simulink model "system_model"  (R2025b)
settings: Solver=FixedStepAuto  StartTime=0.0  StopTime=10  FixedStep=t_s  RelTol=1e-3
values from neighbouring files (symbols this model uses):
  D = Cpid.Kd    [system_init.m]
  denom = [I*L I*R (L*c + k_f*k_e*r^2)  R*c]    [system_init.m]
  I_ = Cpid.Ki    [system_init.m]
  k_enc = 4096 / (2 * pi)    (= 651.898646904)    [system_init.m]
  N = 1/Cpid.Tf    [system_init.m]
  nom = r*k_f    (= 0.73794)    [system_init.m]
  P = Cpid.Kp    [system_init.m]
  r_2 = r    (= 0.1004)    [system_init.m]
  t_s = 0.0005    [system_init.m]
  V_max = 60    [system_init.m]
libraries: slpidlib x1
settings Model: Creator=KnaZ  LastModifiedBy=KnaZ

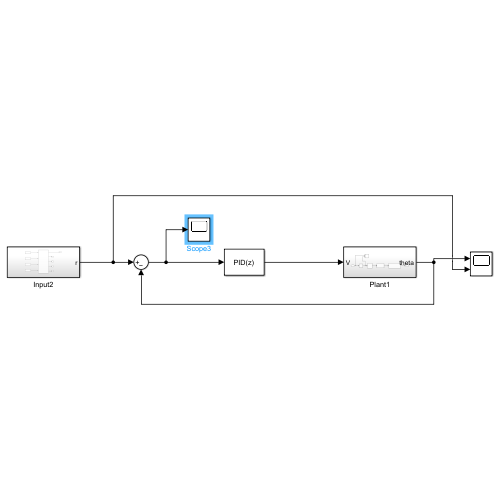
[thumbnail: Simulink's stored preview of the top-level diagram]
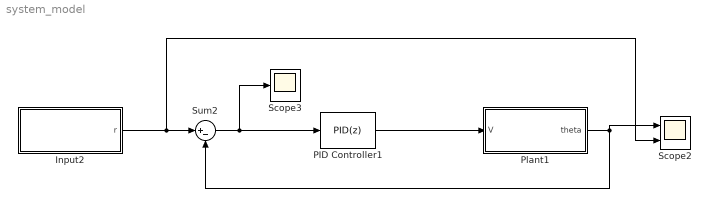
== system system_model ==
  Input2 : Subsystem
  PID Controller1 : slpidlib/PID Controller  Controller=PID  Form=Ideal  TimeDomain=Discrete-time  UseExternalTs=off  SampleTime=t_s  IntegratorMethod=Forward Euler  FilterMethod=Forward Euler  ControllerParametersSource=internal  P=P/10  I=I_  UseKiTs=off  D=D  UseExternalDerivativeSource=off  N=N  UseFilter=on  TunerSelectOption=Transfer Function Based (PID Tuner App)  InitialConditionSource=internal  InitialConditionForIntegrator=0  InitialConditionForFilter=0  DifferentiatorICPrevScaledInput=0  ExternalReset=none  TrackingMode=off  Kt=I_  LimitOutput=off  SatLimitsSource=internal  UpperSaturationLimit=60  LowerSaturationLimit=-60  LinearizeAsGain=off  AntiWindupMode=clamping  Kb=1  LimitIntegrator=off  UpperIntegratorSaturationLimit=inf  LowerIntegratorSaturationLimit=-inf  POutMin=[]  POutMax=[]  IOutMin=[]  IOutMax=[]  DOutMin=[]  DOutMax=[]  NOutMin=[]  NOutMax=[]  SumOutMin=[]  SumOutMax=[]  SaturationOutMin=[]  SaturationOutMax=[]  PParamMin=[]  PParamMax=[]  IParamMin=[]  IParamMax=[]  DParamMin=[]  DParamMax=[]  NParamMin=[]  NParamMax=[]  KbParamMin=[]  KbParamMax=[]  KtParamMin=[]  KtParamMax=[]  KbOutMin=[]  KbOutMax=[]  KtOutMin=[]  KtOutMax=[]  IntegratorOutMin=[]  IntegratorOutMax=[]  FilterOutMin=[]  FilterOutMax=[]  SumI1OutMin=[]  SumI1OutMax=[]  SumI2OutMin=[]  SumI2OutMax=[]  SumI3OutMin=[]  SumI3OutMax=[]  SumI4OutMin=[]  SumI4OutMax=[]  SumDOutMin=[]  SumDOutMax=[]  DifferentiatorOutMin=[]  DifferentiatorOutMax=[]  FilterDiffOutCoefMin=[]  FilterDiffOutCoefMax=[]  ReciprocalOutMin=[]  ReciprocalOutMax=[]  SumDenOutMin=[]  SumDenOutMax=[]  SumNumOutMin=[]  SumNumOutMax=[]  DivideOutMin=[]  DivideOutMax=[]  UdiffTsProdOutMin=[]  UdiffTsProdOutMax=[]  NTsProdOutMin=[]  NTsProdOutMax=[]  UintegralTsProdOutMin=[]  UintegralTsProdOutMax=[]  UngainTsProdOutMin=[]  UngainTsProdOutMax=[]  ClampingZeroOutDataTypeStr=Inherit: Inherit via back propagation  ClampingZeroOutMin=[]  ClampingZeroOutMax=[]  FilterDenConstantOutDataTypeStr=Inherit: Inherit via back propagation  FilterDenConstantOutMin=[]  FilterDenConstantOutMax=[]  PCopyOutDataTypeStr=Inherit: Inherit via back propagation  PCopyOutMin=[]  PCopyOutMax=[]  NCopyOutDataTypeStr=Inherit: Inherit via back propagation  NCopyOutMin=[]  NCopyOutMax=[]  IntegratorContinuousStateAttributes=''  IntegratorStateMustResolveToSignalObject=off  IntegratorRTWStateStorageClass=Auto  FilterContinuousStateAttributes=''  FilterStateMustResolveToSignalObject=off  FilterRTWStateStorageClass=Auto  ParallelPVariant=Passthrough  IdealPVariant=InternalParameters  IVariant=InternalParameters  DVariant=InternalParameters  IntegratorVariant=Discrete  SatVariant=Disabled  AWVariant=Passthrough  PCopyVariant=Disabled  TRVariant=Disabled  FdbkBlocksVariant=Forward  IdealPFdbkVariant=Disabled  SatFdbkVariant=Disabled  DerivativeFilterVariant=ForwardEulerFilter  NVariant=InternalParameters  NCopyVariant=Disabled  FilterICVariant=InternalICsFilter  IntegratorICVariant=InternalICs  ExternalResetVariant=Disabled  TRSumVariant=Passthrough  SumFdbkVariant=Disabled  SumVariant=Sum_PID  TsampFilterVariant=InternalTs  TsampNgainVariant=Passthrough  TsampIntegralVariant=Disabled_SignalSpec  ExternalSaturationOutDataTypeStr=Inherit: Same as second input  DerivativeSourceVariant=ErrorSignal  PreIntVariant=InternalPreInt
  Plant1 : Subsystem
  Scope2 : Scope  NumInputPorts=2
      settings: ActiveDisplayYMinimum=-0.020443518010116426  ActiveDisplayYMaximum=-0.0090093721690085588
  Scope3 : Scope
      settings: ActiveDisplayYMinimum=-0.0045939575455967042  ActiveDisplayYMaximum=0.0022798434903788887  DataLoggingVariableName=ScopeData2
  Sum2 : Sum  Inputs=|+-
  wires:
  Input2/1(r) -> Scope2/2, Sum2/1
  Plant1/1(theta) -> Scope2/1, Sum2/2
  PID Controller1/1 -> Plant1/1(V)
  Sum2/1 -> Scope3/1, PID Controller1/1

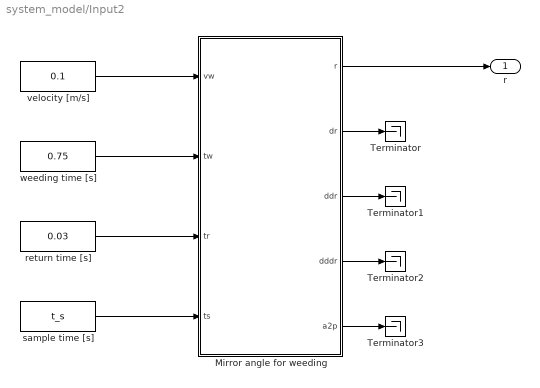
== system system_model/Input2 ==
  Mirror angle for weeding : MATLAB Function  TreatAsAtomicUnit=on
  Terminator{,1..3} (4 alike) : Terminator
  return time [s] : Constant  Value=0.03  SampleTime=t_s
  sample time [s] : Constant  Value=t_s  SampleTime=t_s
  velocity [m/s] : Constant  Value=0.1  SampleTime=t_s
  weeding time [s] : Constant  Value=0.75  SampleTime=t_s
  r : Outport
  wires:
  Mirror angle for weeding/3(ddr) -> Terminator1/1
  Mirror angle for weeding/4(dddr) -> Terminator2/1
  Mirror angle for weeding/1(r) -> r/1
  sample time [s]/1 -> Mirror angle for weeding/4(ts)
  Mirror angle for weeding/2(dr) -> Terminator/1
  return time [s]/1 -> Mirror angle for weeding/3(tr)
  weeding time [s]/1 -> Mirror angle for weeding/2(tw)
  velocity [m/s]/1 -> Mirror angle for weeding/1(vw)
  Mirror angle for weeding/5(a2p) -> Terminator3/1

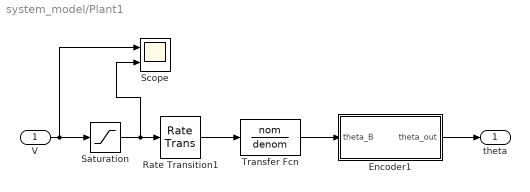
== system system_model/Plant1 ==
  V : Inport
  Encoder1 : Subsystem
  Rate Transition1 : RateTransition  OutPortSampleTime=0
  Saturation : Saturate  UpperLimit=V_max  LowerLimit=-V_max
  Scope : Scope  NumInputPorts=2
      settings: ActiveDisplayYMinimum=-94.384761555803735  ActiveDisplayYMaximum=107.07366746963213  DataLoggingVariableName=ScopeData3
  Transfer Fcn : TransferFcn  Numerator=nom  Denominator=denom
  theta : Outport
  wires:
  Encoder1/1(theta_out) -> theta/1
  V/1 -> Scope/1, Saturation/1
  Saturation/1 -> Scope/2, Rate Transition1/1
  Transfer Fcn/1 -> Encoder1/1(theta_B)
  Rate Transition1/1 -> Transfer Fcn/1

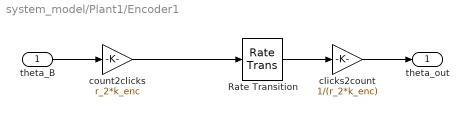
== system system_model/Plant1/Encoder1 ==
  theta_B : Inport
  Rate Transition : RateTransition  OutPortSampleTime=t_s
  clicks2count : Gain  Gain=1/(r_2*k_enc)
  count2clicks : Gain  Gain=r_2*k_enc
  theta_out : Outport
  wires:
  theta_B/1 -> count2clicks/1
  Rate Transition/1 -> clicks2count/1
  clicks2count/1 -> theta_out/1
  count2clicks/1 -> Rate Transition/1

== matlab function system_model/Input2/Mirror angle for weeding ==
  data: vw input; tw input; tr input; r output; dr output; ddr output; dddr output; ts input; a2p output
function [r, dr, ddr, dddr, a2p]   = Trajectory(vw, tw, tr, ts)
% Generates the mirror angle trajectory for weeding

% OUTPUTS:
% reference trajectory
% r:       [rad]     angle
% dr:      [rad/s]   angular velocity 
% ddr:     [rad/s^2] angular acceleration
% dddr:    [rad/s^3] angular jerk
% a2p:     [m/rad]   angle to position transmission

% INPUTS
% vw:       [m/s]   driving velocity
% tw:       [s]     weeding time
% tr:       [s]     return time
% ts:       [s]     sample time

% define time 
persistent t
if isempty(t)
    t = 0;
end
% update time
t = mod(t+ts,tw+tr);  % [s] time
at = 2*pi/tr*t;       % [1/s] angle in period

% auxiliary variables
D = vw*(tw+tr);    % [m] maximum spot amplitude
xs = (D*tw)/(2*(tr + tw)) + (D*(1 - tw^2/(tr + tw)^2)^(1/2))/(2*pi) - (D*tw*acos(tw/(tr + tw)))/(2*pi*(tr + tw)); % [m] maximum amplitude
a2p = xs/17.5e-3;  % [m] angle to position transmission
Da = D/a2p;        % [rad] angular amplitude
va = vw/a2p;       % [rad/s] angular velocity

a = Da*tw/(tw+tr)/2; % [m] polynomial offset cofficient
b = -2*a/tr;         % [m/s] polynomial slope coefficient
c = Da/(2*pi);       % [m] sinusoidal amplitude

% compute angular trajectory and time derivatives
if t <= tr
    % sinusoidal return part
    r       = a+b*t+c*sin(at);
    dr      = b + c*2*pi/tr*cos(at);
    ddr     = -c*(2*pi/tr)^2*sin(at);
    dddr    = -c*(2*pi/tr)^3*cos(at);
else
    % constant velocity welding part
    r       = -Da*tw/(tw+tr)/2+(t-tr)*va;
    dr      = va;
    ddr     = 0;
    dddr    = 0;
end
